simulink model "mgs_multi"  (R2025b)
settings: Solver=ode45  StartTime=0.0  StopTime=50  MaxStep=0.005  RelTol=1e-8  AbsTol=1e-10
undefined symbols (not defined in the file): mgs_N, mgs_X0
settings Model: Creator=joy46  LastModifiedBy=joy46

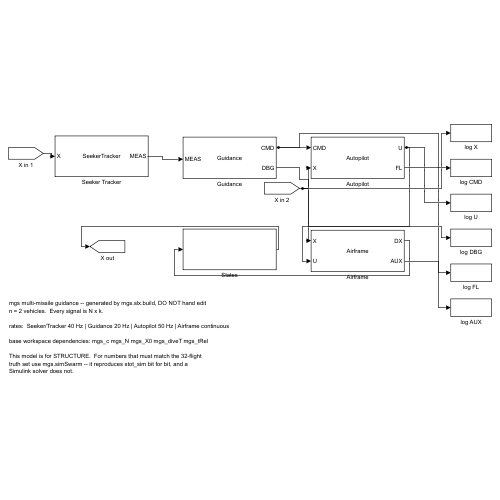
[thumbnail: Simulink's stored preview of the top-level diagram]
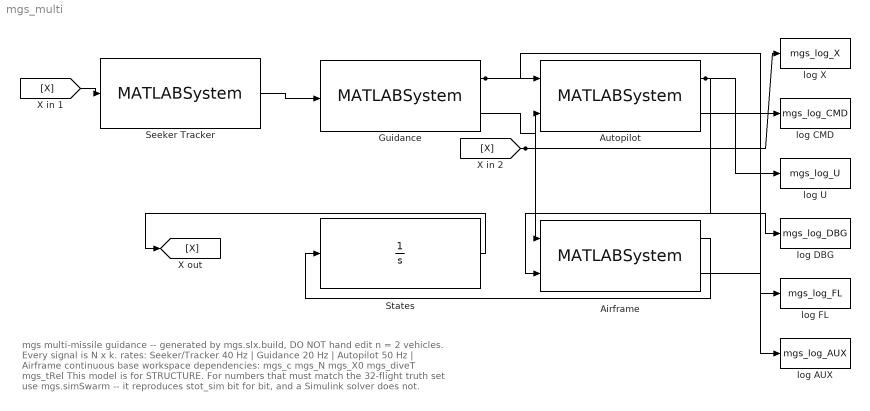
== system mgs_multi ==
  note: mgs multi-missile guidance -- generated by mgs.slx.build, DO NOT hand edit
      | n = 2 vehicles.  Every signal is N x k.
      |
      | rates:  Seeker/Tracker 40 Hz | Guidance 20 Hz | Autopilot 50 Hz | Airframe continuous
      |
      | base workspace dependencies: mgs_c mgs_N mgs_X0 mgs_diveT mgs_tRel
      |
      | This model is for STRUCTURE.  For numbers that must match the 32-flight
      | truth set use mgs.simSwarm -- it reproduces stot_sim bit for bit, and a
      | Simulink solver does not.
  Airframe : MATLABSystem  System=mgs.slx.Airframe  Params=mgs_c  N=mgs_N  SimulateUsing=Interpreted execution
      mask Type: mgs.slx.Airframe
  Autopilot : MATLABSystem  System=mgs.slx.Autopilot  Params=mgs_c  N=mgs_N  SampleTime=0.02  SimulateUsing=Interpreted execution
      mask Type: mgs.slx.Autopilot
  Guidance : MATLABSystem  System=mgs.slx.Guidance  Params=mgs_c  N=mgs_N  SampleTime=0.05  DiveT=mgs_diveT  TRelease=mgs_tRel  SimulateUsing=Interpreted execution
      mask Type: mgs.slx.Guidance
  Seeker Tracker : MATLABSystem  System=mgs.slx.SeekerTracker  Params=mgs_c  N=mgs_N  SampleTime=0.025  SimulateUsing=Interpreted execution
      mask Type: mgs.slx.SeekerTracker
  States : Integrator  InitialCondition=mgs_X0
  log AUX : ToWorkspace  VariableName=mgs_log_AUX  SaveFormat=Structure With Time  SampleTime=-1
  log CMD : ToWorkspace  VariableName=mgs_log_CMD  SaveFormat=Structure With Time  SampleTime=-1
  log DBG : ToWorkspace  VariableName=mgs_log_DBG  SaveFormat=Structure With Time  SampleTime=-1
  log FL : ToWorkspace  VariableName=mgs_log_FL  SaveFormat=Structure With Time  SampleTime=-1
  log U : ToWorkspace  VariableName=mgs_log_U  SaveFormat=Structure With Time  SampleTime=-1
  log X : ToWorkspace  VariableName=mgs_log_X  SaveFormat=Structure With Time  SampleTime=-1
  wires:
  [X] -> Seeker Tracker/1
  Seeker Tracker/1 -> Guidance/1
  Guidance/1 -> Autopilot/1, log CMD/1
  [X] -> Autopilot/2, Airframe/1, log X/1
  Autopilot/1 -> Airframe/2, log U/1
  Airframe/1 -> States/1
  States/1 -> [X]
  Guidance/2 -> log DBG/1
  Autopilot/2 -> log FL/1
  Airframe/2 -> log AUX/1
